simulink model "VoltageDetection_Harness1"  (R2024b)
settings: Solver=VariableStepAuto  StartTime=0.0  StopTime=2  RelTol=1e-3
settings Model: DataDictionary=VoltageDetection.sldd  Creator=User  LastModifiedBy=User

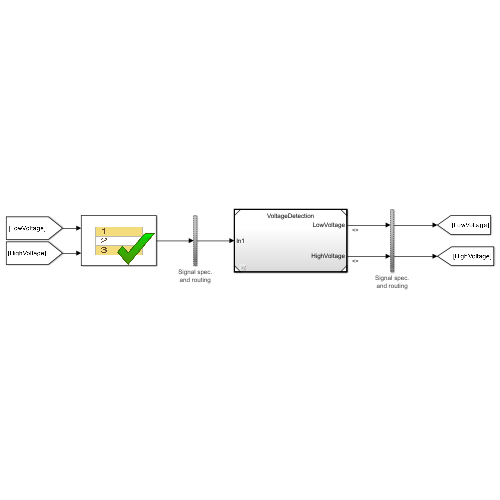
[thumbnail: Simulink's stored preview of the top-level diagram]
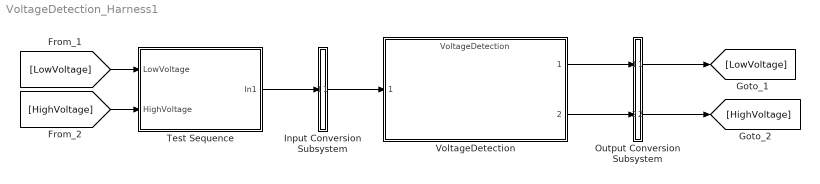
== system VoltageDetection_Harness1 ==
  Input Conversion Subsystem : Subsystem  Tag=__SLT_ICS__  Description=|
      | Signal spec.
      | and routing
      settings: AttributesFormatString=%<Description>
  Output Conversion Subsystem : Subsystem  Tag=__SLT_OCS__  Description=|
      | Signal spec.
      | and routing
      settings: AttributesFormatString=%<Description>
  Test Sequence : Test Sequence  TreatAsAtomicUnit=on
  VoltageDetection : ModelReference  ModelNameDialog=VoltageDetection  SimulationMode=Normal  ModelReferenceVersion=1.7
  wires:
  Test Sequence/1(In1) -> Input Conversion Subsystem/1(Inport_1)
  [LowVoltage] -> Test Sequence/1(LowVoltage)
  [HighVoltage] -> Test Sequence/2(HighVoltage)
  Output Conversion Subsystem/1(Outport_1) -> [LowVoltage]
  Output Conversion Subsystem/2(Outport_2) -> [HighVoltage]
  Input Conversion Subsystem/1(Outport_1) -> VoltageDetection/1
  VoltageDetection/1 -> Output Conversion Subsystem/1(Inport_1)
  VoltageDetection/2 -> Output Conversion Subsystem/2(Inport_2)

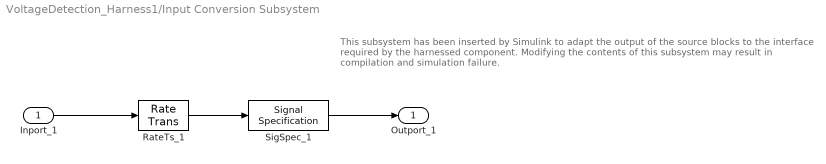
== system VoltageDetection_Harness1/Input Conversion Subsystem ==
  note: This subsystem has been inserted by Simulink to adapt the output of the source blocks to the interface required by the harnessed component.
      |  Modifying the contents of this subsystem may result in compilation and simulation failure.
  Inport_1 : Inport
  RateTs_1 : RateTransition  OutPortSampleTime=0.001
  SigSpec_1 : SignalSpecification  OutDataTypeStr=double  Dimensions=[1]  SampleTime=0.001
  Outport_1 : Outport
  wires:
  SigSpec_1/1 -> Outport_1/1
  RateTs_1/1 -> SigSpec_1/1
  Inport_1/1 -> RateTs_1/1

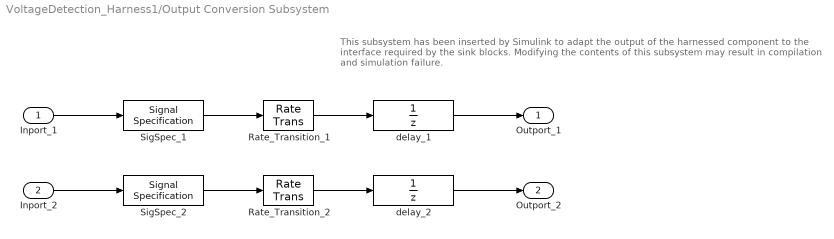
== system VoltageDetection_Harness1/Output Conversion Subsystem ==
  note: This subsystem has been inserted by Simulink to adapt the output of the harnessed component to the interface required by the sink blocks.
      |  Modifying the contents of this subsystem may result in compilation and simulation failure.
  Inport_1 : Inport
  Inport_2 : Inport  Port=2
  Rate_Transition_1 : RateTransition  OutPortSampleTimeOpt=Inherit
  Rate_Transition_2 : RateTransition  OutPortSampleTimeOpt=Inherit
  SigSpec_1 : SignalSpecification  OutDataTypeStr=boolean  Dimensions=[1]  SampleTime=0.001
  SigSpec_2 : SignalSpecification  OutDataTypeStr=boolean  Dimensions=[1]  SampleTime=0.001
  delay_1 : UnitDelay  SampleTime=-1
  delay_2 : UnitDelay  SampleTime=-1
  Outport_1 : Outport
  Outport_2 : Outport  Port=2
  wires:
  Inport_1/1 -> SigSpec_1/1
  SigSpec_1/1 -> Rate_Transition_1/1
  Rate_Transition_1/1 -> delay_1/1
  delay_1/1 -> Outport_1/1
  Inport_2/1 -> SigSpec_2/1
  SigSpec_2/1 -> Rate_Transition_2/1
  Rate_Transition_2/1 -> delay_2/1
  delay_2/1 -> Outport_2/1

== stateflow chart VoltageDetection_Harness1/Test Sequence ==
  state Scenario_1_LowVoltage
    state Run
      %% Initialize data outputs.
      In1 = 260;
    state step_1
      In1 = 0;
    state step_2
      In1 = 1;
    state step_3
      In1 = 150;
    (default) -> Scenario_1_LowVoltage.Run
    Scenario_1_LowVoltage.Run -> Scenario_1_LowVoltage.step_1 : [
        | after(10,msec)
        | ]
    Scenario_1_LowVoltage.step_1 -> Scenario_1_LowVoltage.step_2 : [
        | after(10,msec)
        | ]
    Scenario_1_LowVoltage.step_2 -> Scenario_1_LowVoltage.step_3 : [
        | after(10,msec)
        | ]
  state Scenario_1_HighVoltage
    state Run
      %% Initialize data outputs.
      In1 = 0;
    state step_1
      In1 = 260;
    state step_2
      In1 = 270;
    state step_3
      In1 = 150;
    (default) -> Scenario_1_HighVoltage.Run
    Scenario_1_HighVoltage.Run -> Scenario_1_HighVoltage.step_1 : [
        | after(10,msec)
        | ]
    Scenario_1_HighVoltage.step_1 -> Scenario_1_HighVoltage.step_2 : [
        | after(10,msec)
        | ]
    Scenario_1_HighVoltage.step_2 -> Scenario_1_HighVoltage.step_3 : [
        | after(10,msec)
        | ]
  state Scenario_1_High_Low
    state Run
      %% Initialize data outputs.
      In1 = 150;
    state step_1
      In1 = 260;
    state step_2
      In1 = 0;
    state step_3
      In1 = 1;
    state step_4
      In1 = 260;
    state step_5
      In1 = 2;
    state step_6
      In1 = 1;
    state step_7
      In1 = 150;
    state step_8
      In1 = 150;
    (default) -> Scenario_1_High_Low.Run
    Scenario_1_High_Low.Run -> Scenario_1_High_Low.step_1 : [
        | after(10,msec)
        | ]
    Scenario_1_High_Low.step_1 -> Scenario_1_High_Low.step_2 : [
        | after(20,msec)
        | ]
    Scenario_1_High_Low.step_2 -> Scenario_1_High_Low.step_3 : [
        | after(10,msec)
        | ]
    Scenario_1_High_Low.step_3 -> step_4 : [
        | after(10,msec)
        | ]
    step_4 -> step_5 : [
        | after(10,msec)
        | ]
    step_5 -> step_4 : [
        | after(20,msec)
        | ]
    step_6 -> step_7 : [
        | after(20,msec)
        | ]
    step_7 -> step_8 : [
        | after(20,msec)
        | ]
  (default) -> Scenario_1_LowVoltage [order 1] : [Active_Scenario_Index == 1]
  (default) -> Scenario_1_HighVoltage [order 2] : [Active_Scenario_Index == 2]
  (default) -> Scenario_1_High_Low [order 3] : {assert(Active_Scenario_Index == 3,'The value of Scenario Parameter ''Active_Scenario_Index'' is not valid. Use the index of the scenario to specify it.')}
  data: LowVoltage input boolean size=[1]; HighVoltage input boolean size=[1]; In1 output double size=[1]; Active_Scenario_Index parameter =3
